simulink model "Controller_damping_cbf_22Franka"  (R2022b)
settings: Solver=FixedStepDiscrete  StartTime=0.0  StopTime=inf  FixedStep=0.001  RelTol=1e-3
PreLoadFcn:
  | set_param(gcs, 'RTWSystemTargetFile', 'franka_emika_panda.tlc');
  | 
  | demos_common_configs();
  | collision_behavior = ones(1,52)*100;
values from neighbouring files (symbols this model uses):
  b_sg = fliplr(B(end, :))    [init_damping_cbf.m]
  cbf_damping_params = [cbf_p_ths; cbf_v_ths; cbf_v_0; cbf_gamma; cbf_d_max;                        cbf_w_lin; cbf_w_quad; plane_normal; plane_offset;                        cbf_latch_entry; cbf_zone_hyst; cbf_latch_alpha; cbf_clip_drift;                        cbf_tau_rate; cbf_dt; cbf_gamma_pos_scale]    [init_damping_cbf.m]
  cbf_kappa = 0.85 * cbf_d_max / cbf_rho_eff    (= 82.6388888889)    [init_damping_cbf.m]
  cbf_stiff_decouple = 0    [init_damping_cbf.m]
  Dn = 20 * ones(7,1)    [init_damping_cbf.m]
  H_home = getTransform(Franka_robot, q_home, 'panda_link8', 'panda_link0')    [init_damping_cbf.m]
  Kn = 0 * ones(7,1)    [init_damping_cbf.m]
  plane_normal = [0.0; 0.0; 1.0]    [init_damping_cbf.m]
  q_home = q_init    [init_damping_cbf.m]
  q_init = [0 0  0  -(2/4)*pi  0  pi/2  -pi/4]'    [init_damping_cbf.m]
undefined symbols (not defined in the file or in its folder): DiscIntNeverNeededParam, Fext_mag
libraries: matrix_library x3, franka_simulink_library x2, Robotics_lib x1
(part 1 of 8)
settings Model: SimulationMode=external  ExtModeTrigDuration=10000  Creator=vasi_ko  LastModifiedBy=rsladmin
settings SolverCC: AlgebraicLoopSolver=TrustRegion
settings DataIOCC: LimitDataPoints=on  SaveFormat=Array  ReturnWorkspaceOutputs=off
settings OptimizationCC: EnhancedBackFolding=on  OptimizeBlockOrder=speed  DifferentSizesBufferReuse=on  OptimizationCustomize=off
settings DebuggingCC: SolverPrmCheckMsg=warning  ParameterTunabilityLossMsg=error  UnconnectedInputMsg=warning  UnconnectedOutputMsg=warning  UnconnectedLineMsg=warning  SFUnexpectedBacktrackingDiag=warning  SFNoUnconditionalDefaultTransitionDiag=warning  SFExecutionAtInitializationDiag=none  SFMachineParentedDataDiag=warning  ArithmeticOperatorsInVariantConditions=warning
settings HardwareCC: ProdBitPerLong=64  ProdHWDeviceType=Intel->x86-64 (Linux 64)
settings ModelReferenceCC: EnableRefExpFcnMdlSchedulingChecks=on  PropagateSignalLabelsOutOfModel=off
settings SFSimCC: SimUseLocalCustomCode=off  MATLABDynamicMemAlloc=off  CustomCodeUndefinedFunction=UseInterfaceOnly  SimTargetLang=C++
settings RTWCC: SystemTargetFile=franka_emika_panda.tlc  RTWUseLocalCustomCode=off  Toolchain=Franka Simulink | gmake (64-bit linux)  BuildConfiguration=Faster Runs  TargetLang=C++
settings RTWCC: CustomSource=|
  | /home/rsladmin/employees/parma/cbf_kinteach/damping_cbf_controller/src/damping_cbf_controller.cpp
  | /home/rsladmin/employees/parma/cbf_kinteach/cbf_common/src/profiles.cpp
settings CodeAppCC: OperatorAnnotations=on
settings STFCustomTargetCC: TargetLangStandard=C99 (ISO)  ModelReferenceCompliant=off  MatFileLogging=on  GRTInterface=on  UseToolchainInfoCompliant=on  SystemTargetFile=franka_emika_panda.tlc
settings GRTTargetCC: ModelReferenceCompliant=off  ParMdlRefBuildCompliant=off  CompOptLevelCompliant=off  ConcurrentExecutionCompliant=off  CombineOutputUpdateFcns=off  CPPClassGenCompliant=off  GRTInterface=on  ExtModeStaticAlloc=on  ExtModeTransport=1  ExtModeMexFile=ext_xcp  ExtModeIntrfLevel=Level2 - Open
settings ConfigComp: CovMetricSettings=dw  CovSaveCumulativeToWorkspaceVar=on  CovSaveSingleToWorkspaceVar=on  CovExternalEMLEnable=off  CovSFcnEnable=off

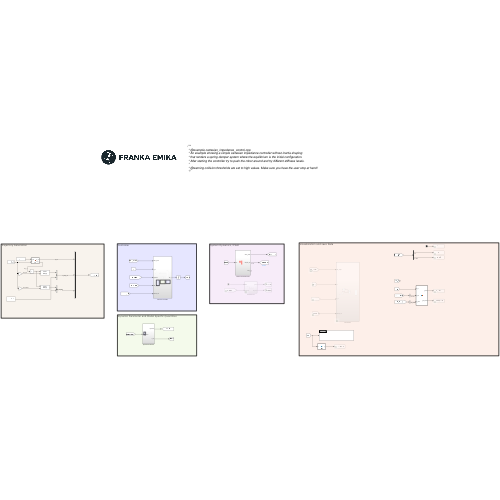
[thumbnail: Simulink's stored preview of the top-level diagram]
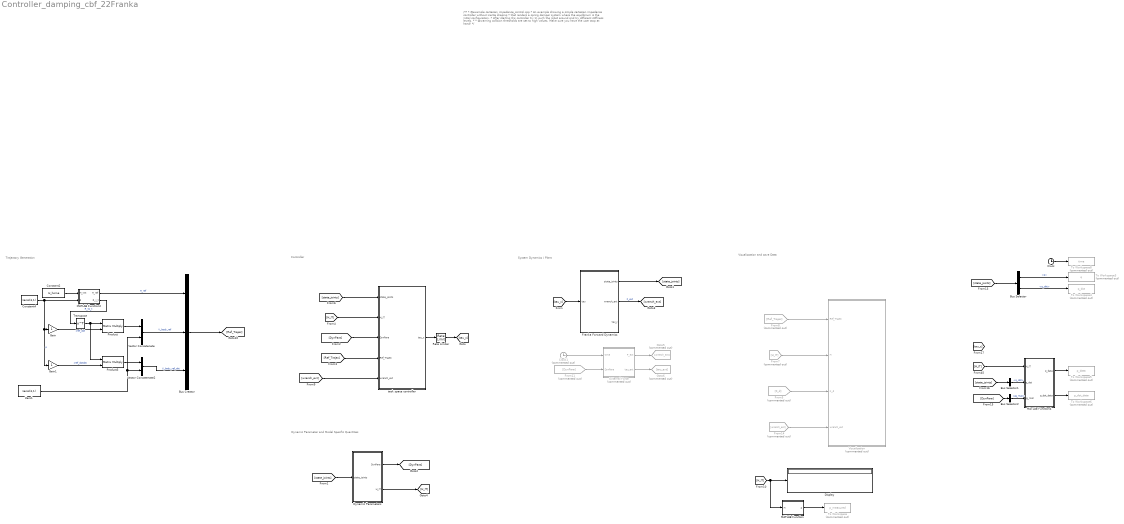
== system Controller_damping_cbf_22Franka ==
  note: /**
      |  * @example cartesian_impedance_control.cpp
      |  * An example showing a simple cartesian impedance controller without inertia shaping
      |  * that renders a spring damper system where the equilibrium is the initial configuration.
      |  * After starting the controller try to push the robot around and try different stiffness levels.
      |  *
      |  * @warning collision thresholds are set to high values. Make sure you have the user stop at hand!
      |  */
  note: Visualiszation and save Data
  note: Dynamic Parameter and Model Specific Quantities
  note: Controller
  note: System Dynamics / Plant
  note: Trajectory Generation
  Bus Creator : BusCreator  Inputs=3
  Bus Selector : BusSelector  OutputSignals=q,q_dot
  Bus Selector1 : BusSelector  OutputSignals=q_dot
  Bus Selector2 : BusSelector  OutputSignals=Jg_mat
  Clock : Clock
  Clock1 : Clock  Commented=on
  Constant2 : Constant  Value=H_home
  Constant4 : Constant  Value=zeros(3,1)
  Display : Display
  Dynamic Parameters : Subsystem
  External Force : Subsystem  Commented=on
  "Franka Forward Dynamics " : Subsystem
  From11 : From  Commented=on  GotoTag=DynPara
  From14 : From  Commented=on  GotoTag=wrench_ext
  From5 : From  Commented=on  GotoTag=K_d
  From7 : From  Commented=on  GotoTag=H_IT
  From8 : From  Commented=on  GotoTag=Ref_Trajec
  Gain : Gain
  Gain1 : Gain
  Goto5 : Goto  Commented=on  GotoTag=wrench_ext
  Goto6 : Goto  Commented=on  GotoTag=tau_ext
  MATLAB Function : MATLAB Function  TreatAsAtomicUnit=on
  MATLAB Function2 : MATLAB Function  TreatAsAtomicUnit=on
  MATLAB Function4 : MATLAB Function  TreatAsAtomicUnit=on
  Product : Product  Multiplication=Matrix(*)
  Product3 : Product  Multiplication=Matrix(*)
  Rate Limiter : RateLimiter  RisingSlewLimit=999  FallingSlewLimit=-999  SampleTimeMode=inherited
  To Workspace : ToWorkspace  Commented=on  VariableName=p_measured  SampleTime=-1
  To Workspace3 : ToWorkspace  Commented=on  VariableName=q  SampleTime=-1
  To Workspace4 : ToWorkspace  Commented=on  VariableName=q_dot  SampleTime=-1
  To Workspace5 : ToWorkspace  Commented=on  VariableName=p_data  SampleTime=-1
  To Workspace6 : ToWorkspace  Commented=on  VariableName=p_dot_data  SampleTime=-1
  To Workspace8 : ToWorkspace  Commented=on  VariableName=time  SampleTime=-1
  Transpose : Math  Operator=transpose
  Vector Concatenate : Concatenate
  Vector Concatenate2 : Concatenate
  Visualisation : Subsystem  Commented=on
  Zero1 : Constant  Value=zeros(3,1)  OutDataTypeStr=Inherit: Inherit via back propagation
  task space controller : Subsystem
  wires:
  From11/1 -> External Force/2(DynPara)
  [state_joints] -> task space controller/1(state_joints)
  Bus Selector/1 -> To Workspace3/1  "<q>"
  [DynPara] -> Bus Selector2/1
  Clock/1 -> To Workspace8/1
  External Force/2(tau_ext) -> Goto6/1
  From7/1 -> Visualisation/2(H)
  From14/1 -> Visualisation/4(wrench_ext)
  [DynPara] -> task space controller/3(DynPara)
  [H_IT] -> MATLAB Function4/1(H_IT)
  Clock1/1 -> External Force/1(time)
  External Force/1(F_ext) -> Goto5/1
  Bus Selector1/1 -> MATLAB Function4/2(q_dot)  "<q_dot>"
  [state_joints] -> Bus Selector1/1
  Dynamic Parameters/2(H_IT) -> [H_IT]
  From5/1 -> Visualisation/3(K_d)
  Rate Limiter/1 -> [tau_c]
  "Franka Forward Dynamics "/1(state_joints) -> [state_joints]
  task space controller/1(tau_c) -> Rate Limiter/1
  [state_joints] -> Bus Selector/1
  Dynamic Parameters/1(DynPara) -> [DynPara]
  MATLAB Function4/2(p_dot_data) -> To Workspace6/1
  [H_IT] -> task space controller/2(H_IT)
  Bus Selector2/1 -> MATLAB Function4/3(Jg_mat)  "<Jg_mat>"
  [wrench_ext] -> task space controller/5(wrench_ext)
  [Ref_Trajec] -> task space controller/4(Ref_Trajec)
  [H_IT] -> MATLAB Function/1(H), Display/1
  MATLAB Function4/1(p_data) -> To Workspace5/1
  From8/1 -> Visualisation/1(Ref_Trajec)
  MATLAB Function/1(p) -> To Workspace/1
  Bus Selector/2 -> To Workspace4/1  "<q_dot>"
  [state_joints] -> Dynamic Parameters/1(state_joints)
  [tau_c] -> "Franka Forward Dynamics "/1(tau)
  Bus Creator/1 -> [Ref_Trajec]
  Transpose/1 -> Product3/1, Product/1
  Zero1/1 -> Vector Concatenate/2, Vector Concatenate2/2
  Constant2/1 -> MATLAB Function2/1(H_init)
  Product/1 -> Vector Concatenate/1
  Gain1/1 -> Product3/2  "xref_dotdot"
  Vector Concatenate2/1 -> Bus Creator/3  "V_body_ref_dot"
  Constant4/1 -> Gain1/1, Gain/1, MATLAB Function2/2(d)  "p"
  Gain/1 -> Product/2  "xref_dot"
  Vector Concatenate/1 -> Bus Creator/2  "V_body_ref"
  MATLAB Function2/2(R_I_t) -> Transpose/1  "R_ts_t"
  MATLAB Function2/1(H_ref) -> Bus Creator/1  "H_ref"
  Product3/1 -> Vector Concatenate2/1
  "Franka Forward Dynamics "/2(wrench_ext) -> [wrench_ext]  "F_ext"

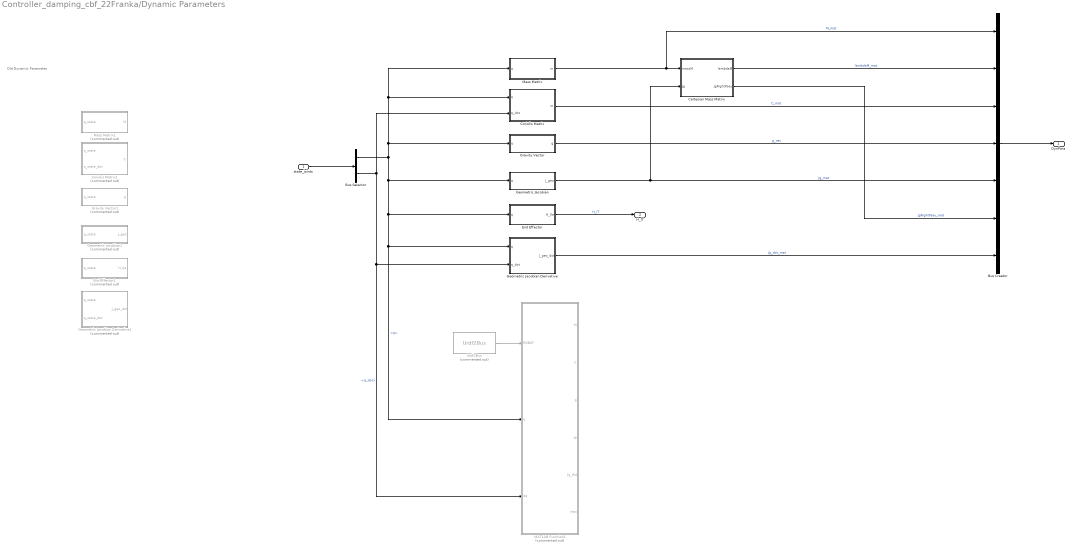
== system Controller_damping_cbf_22Franka/Dynamic Parameters ==
  note: Old Dynamic Parameter
  state_joints : Inport
  Bus Creator : BusCreator  Inputs=7
  Bus Selector : BusSelector  OutputSignals=q,q_dot
  Cartesian Mass Matrix : MATLAB Function  TreatAsAtomicUnit=on
  Coriolis Matrix : MATLAB Function  TreatAsAtomicUnit=on
  Coriolis Matrix1 : MATLAB Function  Commented=on  TreatAsAtomicUnit=on
  End Effector : MATLAB Function  TreatAsAtomicUnit=on
  End Effector1 : MATLAB Function  Commented=on  TreatAsAtomicUnit=on
  Geometric Jacobian : MATLAB Function  TreatAsAtomicUnit=on
  Geometric Jacobian Derivative : MATLAB Function  TreatAsAtomicUnit=on
  Geometric Jacobian Derivative1 : MATLAB Function  Commented=on  TreatAsAtomicUnit=on
  Geometric Jacobian1 : MATLAB Function  Commented=on  TreatAsAtomicUnit=on
  Gravity Vector : MATLAB Function  TreatAsAtomicUnit=on
  Gravity Vector1 : MATLAB Function  Commented=on  TreatAsAtomicUnit=on
  MATLAB Function1 : MATLAB Function  Commented=on  TreatAsAtomicUnit=on
  Mass Matrix : MATLAB Function  TreatAsAtomicUnit=on
  Mass Matrix1 : MATLAB Function  Commented=on  TreatAsAtomicUnit=on
  Urdf2Bus : Robotics_lib/Urdf2Bus  Commented=on  filename='Franka_arm.urdf'  tcp=9  S=[]
  DynPara : Outport
  H_IT : Outport  Port=2
  wires:
  state_joints/1 -> Bus Selector/1
  Urdf2Bus/1 -> MATLAB Function1/1(ROBOT)
  Bus Selector/1 -> Coriolis Matrix/1(q), Mass Matrix/1(q), Gravity Vector/1(q), Geometric Jacobian/1(q), MATLAB Function1/2(q), Geometric Jacobian Derivative/1(q), End Effector/1(q)  "<q>"
  Bus Selector/2 -> Geometric Jacobian Derivative/2(q_dot), MATLAB Function1/3(dq), Coriolis Matrix/2(q_dot)  "<q_dot>"
  Mass Matrix/1(m) -> Bus Creator/1, Cartesian Mass Matrix/1(massM)  "M_mat"
  Bus Creator/1 -> DynPara/1
  Cartesian Mass Matrix/1(lambdaM) -> Bus Creator/2  "lambdaM_mat"
  Coriolis Matrix/1(m) -> Bus Creator/3  "C_mat"
  Gravity Vector/1(g) -> Bus Creator/4  "g_vec"
  Cartesian Mass Matrix/2(JgRightPseu) -> Bus Creator/6  "JgRightPseu_mat"
  Geometric Jacobian Derivative/1(J_geo_dot) -> Bus Creator/7  "Jg_dot_mat"
  End Effector/1(H_0e) -> H_IT/1  "H_IT"
  Geometric Jacobian/1(J_geo) -> Cartesian Mass Matrix/2(Jg), Bus Creator/5  "Jg_mat"

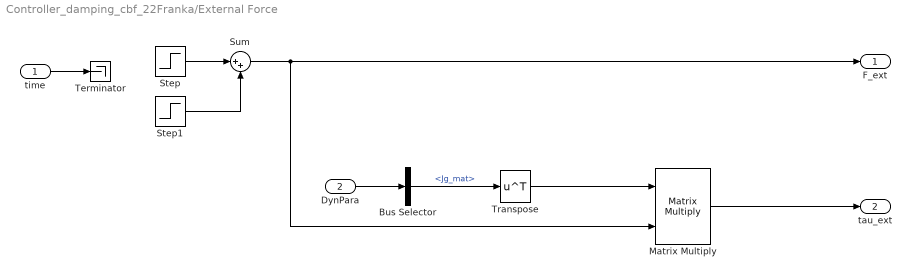
== system Controller_damping_cbf_22Franka/External Force ==
  time : Inport
  DynPara : Inport  Port=2
  Bus Selector : BusSelector  OutputSignals=Jg_mat
  Matrix Multiply : Product  Multiplication=Matrix(*)
  Step : Step  Time=5  Before=zeros(6,1)  After=Fext_mag.*[1;zeros(5,1)]  SampleTime=0
  Step1 : Step  Time=12  Before=zeros(6,1)  After=-Fext_mag.*[1;zeros(5,1)]  SampleTime=0
  Sum : Sum  Inputs=|++
  Terminator : Terminator
  Transpose : Math  Operator=transpose
  F_ext : Outport
  tau_ext : Outport  Port=2
  wires:
  Step/1 -> Sum/1
  Step1/1 -> Sum/2
  time/1 -> Terminator/1
  Sum/1 -> Matrix Multiply/2, F_ext/1
  Transpose/1 -> Matrix Multiply/1
  Bus Selector/1 -> Transpose/1  "<Jg_mat>"
  DynPara/1 -> Bus Selector/1
  Matrix Multiply/1 -> tau_ext/1

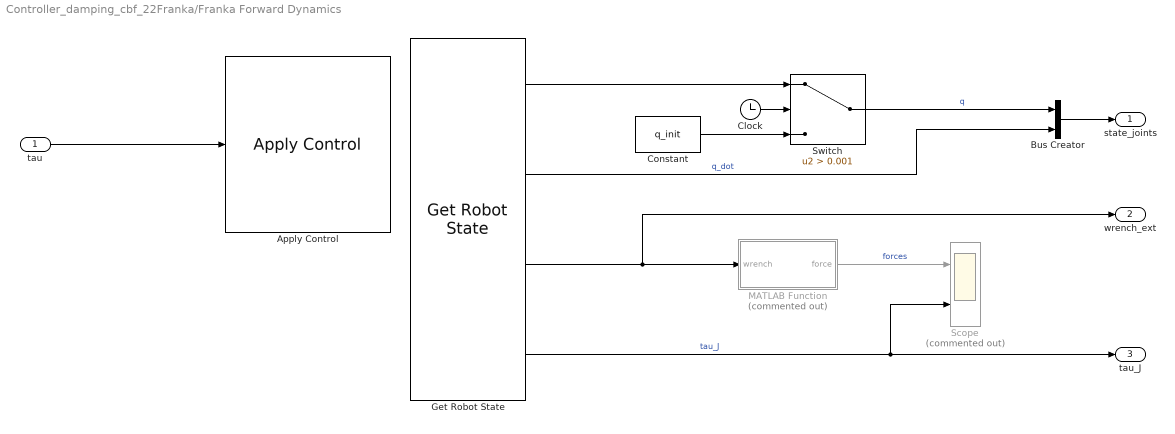
== system Controller_damping_cbf_22Franka/Franka Forward Dynamics  ==
  tau : Inport
  Apply Control : franka_simulink_library/Apply Control  robot_ip=robot_ip  gripper_attached=off  control_mode=Torque Control  controller_choice=Joint Impedance Controller  elbow_control=on  collision_thresholds=100*ones(1,52)  joint_impedance=joint_impedance  cartesian_impedance=cartesian_impedance  load_inertia=load_inertia  EE_T_K=EE_T_K  init_joint_configuration_req=on  init_joint_configuration=q_init'
      settings: SourceProductName=Franka Emika Simulink Support Package
  Bus Creator : BusCreator  Inputs=2
  Clock : Clock
  Constant : Constant  Value=q_init
  Get Robot State : franka_simulink_library/Get Robot State  robot_ip=robot_ip  signals_requested='q dq O_F_ext_hat_K tau_J'
      settings: SourceProductName=Franka Emika Simulink Support Package
  MATLAB Function : MATLAB Function  Commented=on  TreatAsAtomicUnit=on
  Scope : Scope  Commented=on  NumInputPorts=2
  Switch : Switch  Criteria=u2 > Threshold  Threshold=0.001  SaturateOnIntegerOverflow=off  InputSameDT=off
  state_joints : Outport
  wrench_ext : Outport  Port=2
  tau_J : Outport  Port=3
  wires:
  Get Robot State/2 -> Bus Creator/2  "q_dot"
  Get Robot State/1 -> Switch/1
  Get Robot State/3 -> wrench_ext/1, MATLAB Function/1(wrench)
  Constant/1 -> Switch/3
  Switch/1 -> Bus Creator/1  "q"
  Clock/1 -> Switch/2
  MATLAB Function/1(force) -> Scope/1  "forces"
  tau/1 -> Apply Control/1
  Bus Creator/1 -> state_joints/1
  Get Robot State/4 -> tau_J/1, Scope/2  "tau_J"

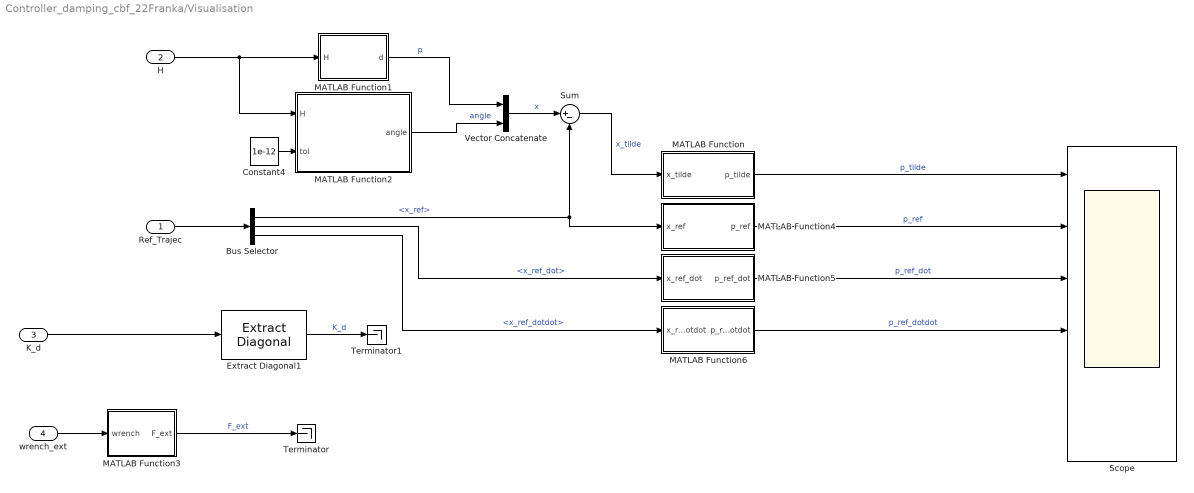
== system Controller_damping_cbf_22Franka/Visualisation ==
  Ref_Trajec : Inport
  H : Inport  Port=2
  K_d : Inport  Port=3
  wrench_ext : Inport  Port=4
  Bus Selector : BusSelector  OutputSignals=x_ref,x_ref_dot,x_ref_dotdot
  Constant4 : Constant  Value=1e-12
  Extract Diagonal1 : matrix_library/Extract Diagonal
      settings: LibrarySourceBlock=|
      | simulink/Matrix
      | Operations/Extract Diagonal
  MATLAB Function : MATLAB Function  TreatAsAtomicUnit=on
  MATLAB Function1 : MATLAB Function  TreatAsAtomicUnit=on
  MATLAB Function2 : MATLAB Function  TreatAsAtomicUnit=on
  MATLAB Function3 : MATLAB Function  TreatAsAtomicUnit=on
  MATLAB Function4 : MATLAB Function  TreatAsAtomicUnit=on
  MATLAB Function5 : MATLAB Function  TreatAsAtomicUnit=on
  MATLAB Function6 : MATLAB Function  TreatAsAtomicUnit=on
  Scope : Scope  NumInputPorts=6
  Sum : Sum  Inputs=|+-
  Terminator : Terminator
  Terminator1 : Terminator
  Vector Concatenate : Concatenate
  wires:
  H/1 -> MATLAB Function2/1(H), MATLAB Function1/1(H)
  MATLAB Function1/1(d) -> Vector Concatenate/1  "p"
  Ref_Trajec/1 -> Bus Selector/1
  Bus Selector/1 -> MATLAB Function4/1(x_ref), Sum/2  "<x_ref>"
  MATLAB Function/1(p_tilde) -> Scope/1  "p_tilde"
  Constant4/1 -> MATLAB Function2/2(tol)
  MATLAB Function2/1(angle) -> Vector Concatenate/2  "angle"
  Vector Concatenate/1 -> Sum/1  "x"
  Sum/1 -> MATLAB Function/1(x_tilde)  "x_tilde"
  Extract Diagonal1/1 -> Terminator1/1  "K_d"
  wrench_ext/1 -> MATLAB Function3/1(wrench)
  MATLAB Function3/1(F_ext) -> Terminator/1  "F_ext"
  K_d/1 -> Extract Diagonal1/1
  MATLAB Function4/1(p_ref) -> Scope/2  "p_ref"
  MATLAB Function5/1(p_ref_dot) -> Scope/3  "p_ref_dot"
  Bus Selector/2 -> MATLAB Function5/1(x_ref_dot)  "<x_ref_dot>"
  MATLAB Function6/1(p_ref_dotdot) -> Scope/4  "p_ref_dotdot"
  Bus Selector/3 -> MATLAB Function6/1(x_ref_dotdot)  "<x_ref_dotdot>"

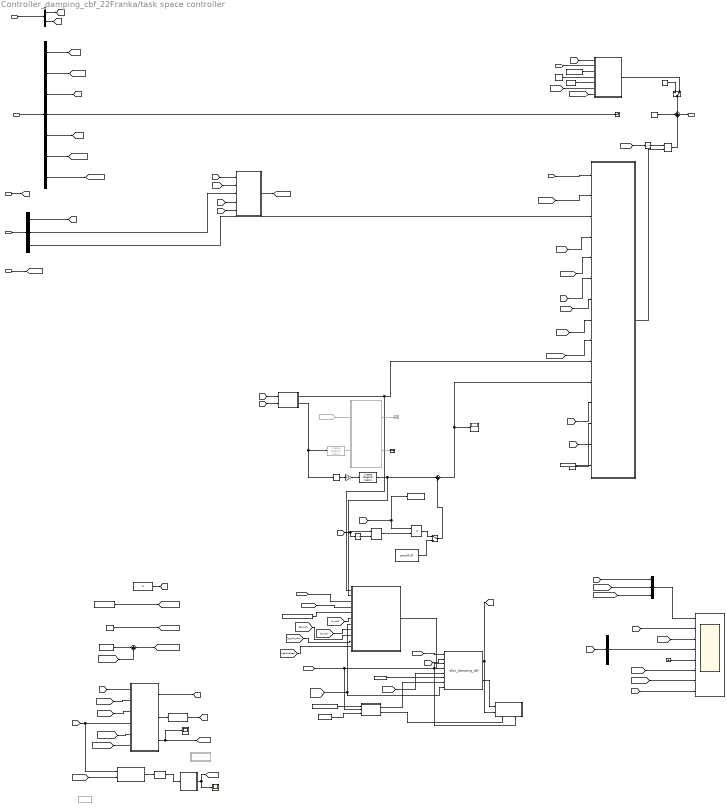
== system Controller_damping_cbf_22Franka/task space controller ==
  note: normalvector of hyperplane
      | + 3 zeros for the angular part
  note: with Box set = 0.106 m
      | regular table without box set = -0.004
      | Box on Table = 0.106-0.004
  note: with Waping endeffector set = 0.055
  note: (1 - x/x0)^expo
  note: 0 = constant
      | 1 = Christian's
      | 2 = My first
      | 3 = General Function
  note: Alt: -2e-3
      | Versuch: -5e-3
  note: 0 = org
      | 1 = moduled
  note: Visualisation
  state_joints : Inport
  H_IT : Inport  Port=2
  DynPara : Inport  Port=3
  Ref_Trajec : Inport  Port=4
  wrench_ext : Inport  Port=5
  Additional_Damping : Constant  Value=70
  Bus Selector : BusSelector  OutputSignals=H_ref,V_body_ref,V_body_ref_dot
  Bus Selector1 : BusSelector  OutputSignals=q,q_dot
  Bus Selector2 : BusSelector  OutputSignals=M_mat,lambdaM_mat,C_mat,g_vec,Jg_mat,JgRightPseu_mat,Jg_dot_mat
  CBF_Telemetry_Visualizer : Subsystem
      settings: PortSchema="{\"entries\":[{\"content\":{\"sides\":[{\"content\":{\"connectorIds\":[\"In1\",\"In2\"]},\"type\":\"ConnectorPlacement.EquallySpacedRectSide\",\"uuid\":\"710f47e5-147d-4a78-88ec-e281af76ee9f\"},{\"content\":{\"connectorIds\":[],\"side\":\"RIGHT\"},\"type\":\"ConnectorPlacement.EquallySpacedRectSide\",\"uuid\":\"9aa80510-4d6e-46c3-afa9-ad1226fbedc7\"},{\"content\":{\"connectorIds\":[],\"side\":\"TOP\"},\"type\":\"ConnectorPlacement.EquallySpacedRectSide\",\"uuid\":\"974fed3d-c6d1-41f4-ba7d-92d951d4e310\"},{\"content\":{\"connectorIds\":[\"In3\",\"In4\"],\"side\":\"BOTTOM\"},\"type\":\"ConnectorPlacement.EquallySpacedRectSide\",\"uuid\":\"a224dcdf-4876-4c61-a8a6-cdf7785f6603\"}]},\"type\":\"ConnectorPlacement.EquallySpacedConnector\",\"uuid\":\"a51230df-76b2-4a69-8099-ddb5762480b7\"}],\"packageUris\":[\"http://schema.mathworks.com/mf0/Connector/R2020b\"],\"version\":\"1.0\"}"
  Compute eff d_max : MATLAB Function  TreatAsAtomicUnit=on
  Compute_F_nominal : MATLAB Function  TreatAsAtomicUnit=on
  Const_StiffDecouple_fnom : Constant  Value=cbf_stiff_decouple
  Const_StiffDecouple_imp : Constant  Value=cbf_stiff_decouple
  Constant : Constant  Value=Dn
  Constant1 : Constant  Commented=on  Value=zeros(3,1)
  Constant10 : Constant  Value=zeros(6,6)
  Constant2 : Constant  Value=cbf_kappa
  Constant3 : Constant  Value=q_home
  Constant4 : Constant  Value=0.*Kn
  Constant7 : Constant  Value=[plane_normal(:)./norm(plane_normal); 0; 0; 0]  VectorParams1D=off
  Constant_cbf_params : Constant  Value=cbf_damping_params
  Constant_use_fext_damp : Constant
  Create Diagonal Matrix : matrix_library/Create Diagonal Matrix  Commented=on
      settings: LibrarySourceBlock=|
      | simulink/Matrix
      | Operations/Create Diagonal
      | Matrix
  Create Diagonal Matrix1 : matrix_library/Create Diagonal Matrix
      settings: LibrarySourceBlock=|
      | simulink/Matrix
      | Operations/Create Diagonal
      | Matrix
  Damping Desing Selection : Subsystem  Commented=on
  Discrete FIR Filter : DiscreteFir  Coefficients=b_sg
  Display : Display
  From1 : From  Commented=on  GotoTag=lambda_mat
  Gain : Gain  Gain=0.6
  Ground_Scope_5 : Ground
  MATLAB Function1 : MATLAB Function  TreatAsAtomicUnit=on
  MATLAB Function15 : MATLAB Function  TreatAsAtomicUnit=on
  MATLAB Function2 : MATLAB Function  TreatAsAtomicUnit=on
  Manual Switch : ManualSwitch  CurrentSetting=0
  Manual Switch1 : ManualSwitch
  MatrixMultiply1 : Product  Multiplication=Matrix(*)
  MatrixMultiply2 : Product  Multiplication=Matrix(*)
  MatrixMultiply3 : Product
  OLD FILTERiNG : Subsystem  Commented=on
  S-Function Damping CBF : S-Function  FunctionName=sfun_damping_cbf  SFunctionDeploymentMode=off  EnableBusSupport=off
  Scope : Scope
  Scope3 : Scope
  Scope:DapingPara1 : Scope  NumInputPorts=8
  Sqrt : Sqrt
  Stiffnessforces : Subsystem
  Subsystem2 : Subsystem
  Subsystem4 : Subsystem
  Sum : Sum  Inputs=+++
  Sum3 : Sum  Inputs=|++
  Sum4 : Sum  Inputs=|+-
  Terminator : Terminator
  Terminator1 : Terminator
  Terminator2 : Terminator  Commented=on
  To Workspace : ToWorkspace  VariableName=d_add  SampleTime=-1
  Transpose : Math  Operator=transpose
  Transpose1 : Math  Operator=transpose
  Vector Concatenate2 : Concatenate  NumInputs=3
  Vector Concatenate3 : Concatenate  NumInputs=1
  Zero : Constant  Value=0  OutDataTypeStr=Inherit: Inherit via back propagation
  Zero1 : Constant  Value=0  OutDataTypeStr=Inherit: Inherit via back propagation
  endEffector_height : Constant  Value=0
  impedance controller1 : MATLAB Function  TreatAsAtomicUnit=on
  nullspace damping : MATLAB Function  TreatAsAtomicUnit=on
  xTableHight : Constant  Value=0.106-0.004
  xthreshold_TSD : Constant  Value=0.30
  tau_c : Outport
  wires:
  state_joints/1 -> Bus Selector1/1
  Sum/1 -> tau_c/1
  Constant/1 -> nullspace damping/5(Dn)
  Bus Selector/1 -> [H_ref]  "<H_ref>"
  Bus Selector/2 -> Subsystem4/3(V_body_ref)  "<V_body_ref>"
  MatrixMultiply1/1 -> Sum/3
  nullspace damping/1(tau_nullspace) -> Manual Switch/2  "tau_null"
  Ref_Trajec/1 -> Bus Selector/1
  Bus Selector/3 -> impedance controller1/3(V_ref_dot)  "<V_body_ref_dot>"
  DynPara/1 -> Bus Selector2/1
  Bus Selector2/1 -> [M_mat]  "<M_mat>"
  Bus Selector2/3 -> [C_mat]  "<C_mat>"
  Bus Selector2/4 -> Terminator1/1  "<g_vec>"
  [q] -> nullspace damping/1(q)
  Bus Selector2/5 -> [Jg_mat]  "<Jg_mat>"
  Bus Selector2/7 -> [Jg_dot_mat]  "<Jg_dot_mat>"
  [Jg_mat] -> nullspace damping/6(Jg)
  Bus Selector2/2 -> [lambda_mat]  "<lambdaM_mat>"
  Constant3/1 -> nullspace damping/3(q_ref)
  Constant4/1 -> nullspace damping/4(Kn)
  Bus Selector2/6 -> [JgRightPseu]  "<JgRightPseu_mat>"
  [JgRightPseu] -> nullspace damping/7(JgRightPseu)
  Bus Selector1/2 -> [q_dot]  "<q_dot>"
  [q_dot] -> nullspace damping/2(q_dot)
  [q_dot] -> impedance controller1/1(q_dot)
  From1/1 -> Damping Desing Selection/1(Lambda_mat)
  Bus Selector1/1 -> [q]  "<q>"
  wrench_ext/1 -> [wrench_ext]
  Zero/1 -> Manual Switch/1
  Create Diagonal Matrix/1 -> Damping Desing Selection/2(Kd)
  Sum3/1 -> impedance controller1/11(Dd), Display/1
  xthreshold_TSD/1 -> Sum4/1
  [V_tilde] -> MATLAB Function2/2(V_tilde)
  [H_IT] -> MATLAB Function2/1(H_IT)
  [lambda_mat] -> MATLAB Function2/3(lambda_mat)
  xTableHight/1 -> [xTableHight]
  MATLAB Function2/1(x_c) -> [x_c]
  Subsystem2/1(x) -> [v_c]  "v_c"
  [q_dot] -> Subsystem4/1(q_dot)
  [Jg_mat] -> Subsystem4/2(Jg)
  Subsystem4/1(V_tilde) -> [V_tilde]
  [V_tilde] -> impedance controller1/2(V_tilde)
  [M_mat] -> impedance controller1/4(massM)
  [lambda_mat] -> impedance controller1/5(lambdaM)
  [C_mat] -> impedance controller1/6(C)
  [Jg_mat] -> impedance controller1/7(Jg)
  [Jg_dot_mat] -> impedance controller1/8(Jg_dot)
  [JgRightPseu] -> impedance controller1/9(JgRightPseu)
  Stiffnessforces/1(Fk) -> impedance controller1/10(Fk), Compute_F_nominal/1(Fk)
  [H_ref] -> Subsystem4/5(H_ref)
  [H_ref] -> Stiffnessforces/2(H_ref)
  [H_ref] -> impedance controller1/12(H_I_D)
  Stiffnessforces/2(K_d) -> Create Diagonal Matrix/1, Sqrt/1
  H_IT/1 -> [H_IT]
  [H_IT] -> Subsystem4/4(Htm)
  [H_IT] -> Stiffnessforces/1(H)
  Damping Desing Selection/1(K_ref) -> Terminator2/1
  Manual Switch/1 -> Sum/1
  endEffector_height/1 -> [eef_height]
  Constant7/1 -> [n_hp]
  MATLAB Function2/3(m_c) -> Scope3/1, [mass_c]
  [n_hp] -> impedance controller1/13(n_hp)
  Additional_Damping/1 -> impedance controller1/14(d_add)
  impedance controller1/1(F_control) -> MatrixMultiply1/2
  [Jg_mat] -> Transpose/1
  Transpose/1 -> MatrixMultiply1/1
  [n_hp] -> MatrixMultiply2/1, Transpose1/1
  Transpose1/1 -> MatrixMultiply2/2
  MatrixMultiply2/1 -> MatrixMultiply3/2
  [damp] -> To Workspace/1, MatrixMultiply3/1
  Sqrt/1 -> Gain/1
  Gain/1 -> Create Diagonal Matrix1/1
  Create Diagonal Matrix1/1 -> Sum3/1, Compute_F_nominal/2(D0)
  [xTableHight] -> MATLAB Function2/5(xTableHight)
  [eef_height] -> MATLAB Function2/6(eef_height)
  [xTableHight] -> Sum4/2
  Sum4/1 -> [xthreshold_TSD]
  Manual Switch1/1 -> Sum3/2
  MATLAB Function2/2(v_c) -> Subsystem2/1(u)  "v_c"
  [x_c] -> Vector Concatenate2/1  "x_c"
  [xthreshold_TSD] -> Vector Concatenate2/3  "xthreshold_TSD"
  Vector Concatenate3/1 -> Scope:DapingPara1/4
  [pointOfIntersec] -> Scope:DapingPara1/7  "pointOfIntersec"
  [x_c_modified] -> Vector Concatenate2/2  "x_c_modified"
  [n_hp] -> Scope:DapingPara1/8  "n_hp"
  Vector Concatenate2/1 -> Scope:DapingPara1/1
  [mass_c] -> Scope:DapingPara1/6
  [v_c] -> Scope:DapingPara1/2  "v_c"
  Damping Desing Selection/2(D_ref) -> Terminator/1
  Constant10/1 -> Manual Switch1/2
  MatrixMultiply3/1 -> Manual Switch1/1
  [F_ext] -> Scope:DapingPara1/3
  Ground_Scope_5/1 -> Scope:DapingPara1/5
  [V_tilde] -> Compute_F_nominal/3(V_tilde)
  [x_c] -> S-Function Damping CBF/1
  [mass_c] -> Compute eff d_max/2(rho), S-Function Damping CBF/3, CBF_Telemetry_Visualizer/4(m_eff)
  Compute_F_nominal/1(F_nominal) -> S-Function Damping CBF/4
  [F_ext] -> S-Function Damping CBF/5
  Constant_use_fext_damp/1 -> S-Function Damping CBF/6
  Constant_cbf_params/1 -> Compute eff d_max/1(params_in)
  S-Function Damping CBF/1 -> [damp], CBF_Telemetry_Visualizer/2(d_cbf)
  S-Function Damping CBF/2 -> CBF_Telemetry_Visualizer/1(telem)
  [v_c] -> S-Function Damping CBF/2
  Zero1/1 -> Sum/2
  MATLAB Function15/1(F) -> Scope/1, [F_ext]
  [n_hp] -> MATLAB Function1/1(n_hp), MATLAB Function2/4(n_hp)
  [wrench_ext] -> MATLAB Function1/2(wrench_ext)
  [damp] -> Vector Concatenate3/1
  Discrete FIR Filter/1 -> MATLAB Function15/1(u)
  MATLAB Function1/1(F_ext) -> Discrete FIR Filter/1
  Compute eff d_max/1(params) -> S-Function Damping CBF/7
  Constant2/1 -> Compute eff d_max/3(kappa)
  Compute eff d_max/2(d_max) -> CBF_Telemetry_Visualizer/3(d_max)
  Const_StiffDecouple_imp/1 -> impedance controller1/15(decouple)
  [n_hp] -> Compute_F_nominal/4(n_hp)
  Const_StiffDecouple_fnom/1 -> Compute_F_nominal/5(decouple)
  [M_mat] -> Compute_F_nominal/6(massM)
  [lambda_mat] -> Compute_F_nominal/7(lambdaM), S-Function Damping CBF/8
  [C_mat] -> Compute_F_nominal/8(C)
  [Jg_mat] -> Compute_F_nominal/9(Jg)
  [Jg_dot_mat] -> Compute_F_nominal/10(Jg_dot)
  [JgRightPseu] -> Compute_F_nominal/11(JgRightPseu)

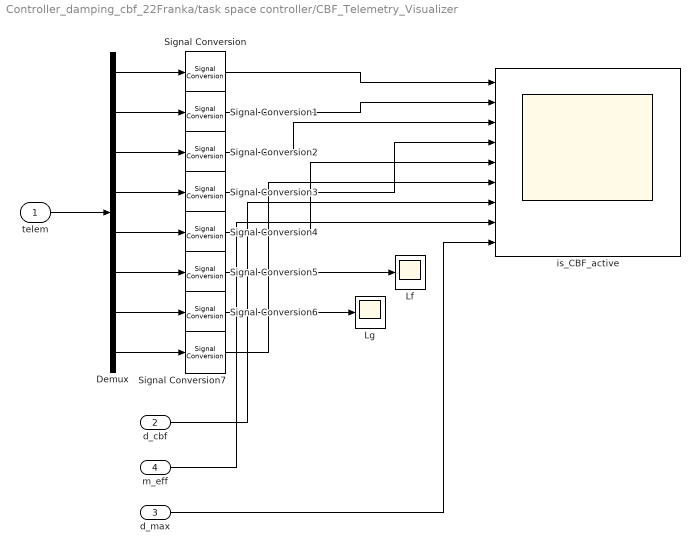
== system Controller_damping_cbf_22Franka/task space controller/CBF_Telemetry_Visualizer ==
  telem : Inport
  d_cbf : Inport  Port=2
  d_max : Inport  Port=3
  m_eff : Inport  Port=4
  Demux : Demux  Outputs=8
  Lf : Scope
  Lg : Scope
  Signal Conversion{,1..7} (8 alike) : SignalConversion  OverrideOpt=off
  is_CBF_active : Scope  NumInputPorts=9
  wires:
  telem/1 -> Demux/1
  Demux/1 -> Signal Conversion/1
  Signal Conversion/1 -> is_CBF_active/1
  Signal Conversion1/1 -> is_CBF_active/2
  Demux/2 -> Signal Conversion1/1
  Signal Conversion2/1 -> is_CBF_active/3
  Demux/3 -> Signal Conversion2/1
  Signal Conversion3/1 -> is_CBF_active/4
  Demux/4 -> Signal Conversion3/1
  Signal Conversion4/1 -> is_CBF_active/5
  Demux/5 -> Signal Conversion4/1
  Signal Conversion5/1 -> Lf/1
  Demux/6 -> Signal Conversion5/1
  Signal Conversion6/1 -> Lg/1
  Demux/7 -> Signal Conversion6/1
  Signal Conversion7/1 -> is_CBF_active/6
  Demux/8 -> Signal Conversion7/1
  d_cbf/1 -> is_CBF_active/7
  m_eff/1 -> is_CBF_active/8
  d_max/1 -> is_CBF_active/9

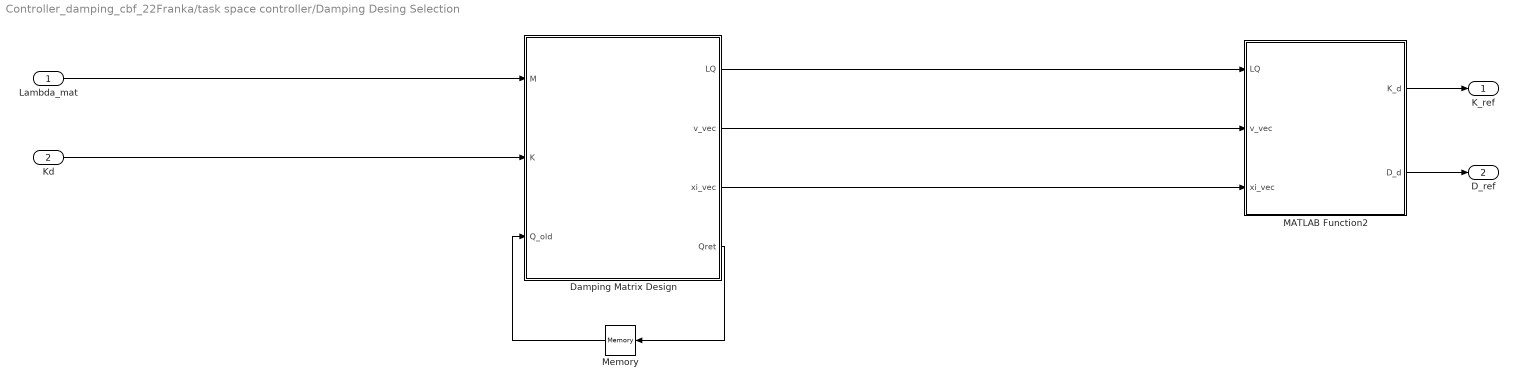
== system Controller_damping_cbf_22Franka/task space controller/Damping Desing Selection ==
  Lambda_mat : Inport
  Kd : Inport  Port=2
  Damping Matrix Design : MATLAB Function  TreatAsAtomicUnit=on
  MATLAB Function2 : MATLAB Function  TreatAsAtomicUnit=on
  Memory : Memory  InitialCondition=eye(6)  InheritSampleTime=on
  K_ref : Outport
  D_ref : Outport  Port=2
  wires:
  Memory/1 -> Damping Matrix Design/3(Q_old)
  Damping Matrix Design/4(Qret) -> Memory/1
  Lambda_mat/1 -> Damping Matrix Design/1(M)
  Damping Matrix Design/3(xi_vec) -> MATLAB Function2/3(xi_vec)
  MATLAB Function2/1(K_d) -> K_ref/1
  MATLAB Function2/2(D_d) -> D_ref/1
  Damping Matrix Design/2(v_vec) -> MATLAB Function2/2(v_vec)
  Damping Matrix Design/1(LQ) -> MATLAB Function2/1(LQ)
  Kd/1 -> Damping Matrix Design/2(K)

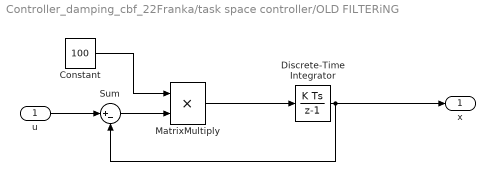
== system Controller_damping_cbf_22Franka/task space controller/OLD FILTERiNG ==
  u : Inport
  Constant : Constant  Value=100
  Discrete-Time Integrator : DiscreteIntegrator  SampleTime=-1  ICPrevOutput=DiscIntNeverNeededParam  ICPrevScaledInput=DiscIntNeverNeededParam
  MatrixMultiply : Product
  Sum : Sum  Inputs=|+-
  x : Outport
  wires:
  u/1 -> Sum/1
  Sum/1 -> MatrixMultiply/2
  Constant/1 -> MatrixMultiply/1
  MatrixMultiply/1 -> Discrete-Time Integrator/1
  Discrete-Time Integrator/1 -> Sum/2, x/1

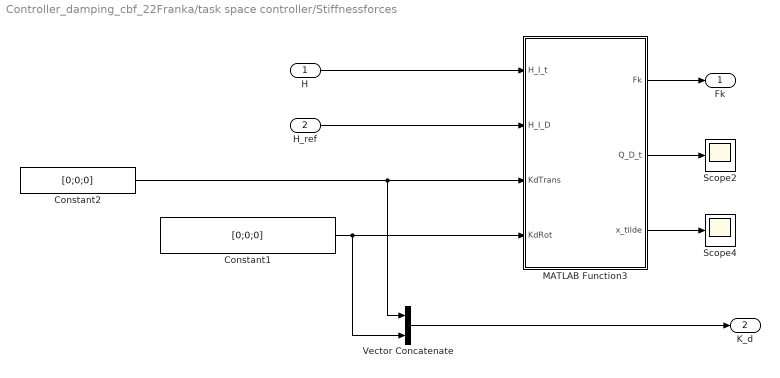
== system Controller_damping_cbf_22Franka/task space controller/Stiffnessforces ==
  H : Inport
  H_ref : Inport  Port=2
  Constant1 : Constant  Value=[0;0;0]
  Constant2 : Constant  Value=[0;0;0]
  MATLAB Function3 : MATLAB Function  TreatAsAtomicUnit=on
  Scope2 : Scope
  Scope4 : Scope
  Vector Concatenate : Concatenate
  Fk : Outport
  K_d : Outport  Port=2
  wires:
  Constant2/1 -> Vector Concatenate/1, MATLAB Function3/3(KdTrans)
  Constant1/1 -> Vector Concatenate/2, MATLAB Function3/4(KdRot)
  H_ref/1 -> MATLAB Function3/2(H_I_D)
  H/1 -> MATLAB Function3/1(H_I_t)
  MATLAB Function3/2(Q_D_t) -> Scope2/1
  MATLAB Function3/3(x_tilde) -> Scope4/1
  MATLAB Function3/1(Fk) -> Fk/1
  Vector Concatenate/1 -> K_d/1

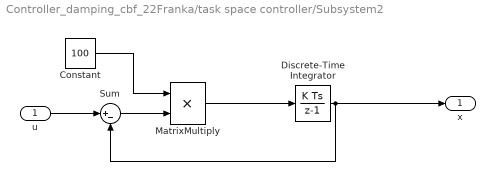
== system Controller_damping_cbf_22Franka/task space controller/Subsystem2 ==
  u : Inport
  Constant : Constant  Value=100
  Discrete-Time Integrator : DiscreteIntegrator  SampleTime=-1  ICPrevOutput=DiscIntNeverNeededParam  ICPrevScaledInput=DiscIntNeverNeededParam
  MatrixMultiply : Product
  Sum : Sum  Inputs=|+-
  x : Outport
  wires:
  u/1 -> Sum/1
  Sum/1 -> MatrixMultiply/2
  Constant/1 -> MatrixMultiply/1
  MatrixMultiply/1 -> Discrete-Time Integrator/1
  Discrete-Time Integrator/1 -> Sum/2, x/1

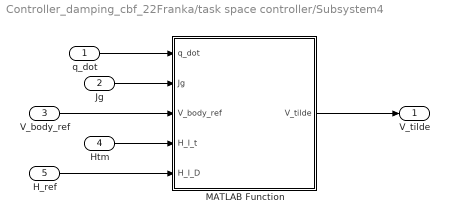
== system Controller_damping_cbf_22Franka/task space controller/Subsystem4 ==
  q_dot : Inport
  Jg : Inport  Port=2
  V_body_ref : Inport  Port=3
  Htm : Inport  Port=4
  H_ref : Inport  Port=5
  MATLAB Function : MATLAB Function  TreatAsAtomicUnit=on
  V_tilde : Outport
  wires:
  MATLAB Function/1(V_tilde) -> V_tilde/1
  Jg/1 -> MATLAB Function/2(Jg)
  q_dot/1 -> MATLAB Function/1(q_dot)
  Htm/1 -> MATLAB Function/4(H_I_t)
  H_ref/1 -> MATLAB Function/5(H_I_D)
  V_body_ref/1 -> MATLAB Function/3(V_body_ref)
